simulink model "Autonomous_Microgrid_Test_backup"  (R2025b)
settings: Solver=FixedStepDiscrete  StartTime=0.0  StopTime=10.0  FixedStep=0.01  RelTol=1e-3  EnableMultiTasking=on
undefined symbols (not defined in the file): I_MAX, T_MAX, V_MAX, V_MIN
libraries: arduinolib x5
settings Model: ExtModeTrigDuration=2  Creator=Faculty  LastModifiedBy=Faculty
settings SolverCC: AutoInsertRateTranBlk=on
settings DataIOCC: ReturnWorkspaceOutputs=off
settings OptimizationCC: EnhancedBackFolding=on  PassReuseOutputArgsAs=Individual arguments  ZeroExternalMemoryAtStartup=off  ZeroInternalMemoryAtStartup=off  MaxStackSize=64  OptimizeBlockOrder=speed  DifferentSizesBufferReuse=on  OptimizationCustomize=off  EfficientTunableParamExpr=on
settings DebuggingCC: ParameterTunabilityLossMsg=error
settings HardwareCC: ProdBitPerPointer=32.0  ProdBitPerSizeT=32.0  ProdBitPerPtrDiffT=32.0  ProdLargestAtomicInteger=Long  ProdLargestAtomicFloat=Double  ProdWordSize=32.0  ProdHWDeviceType=ARM Compatible->ARM Cortex  UseEmbeddedCoderFeatures=off  UseSimulinkCoderFeatures=off
settings SFSimCC: MATLABDynamicMemAlloc=off
settings RTWCC: SystemTargetFile=ert.tlc  HardwareBoard=Arduino Uno R4 WiFi  TemplateMakefile=ert_default_tmf  Toolchain=Arduino ARM M4  BuildConfiguration=Faster Runs  Description=Embedded Coder
settings CodeAppCC: ForceParamTrailComments=on  IgnoreCustomStorageClasses=off  OperatorAnnotations=on  SimulinkDataObjDesc=on  SFDataObjDesc=on  InsertBlockDesc=on
settings ERTTargetCC: ExtModeTransport=3.0  ExtModeStaticAlloc=on  ExtModeAutomaticAllocSize=off  ExtModeStaticAllocSize=8192.0  ExtModeMexFile=ext_xcp  ExtModeIntrfLevel=Level2 - Open  InlinedParameterPlacement=Hierarchical  SupportContinuousTime=on  SupportNonInlinedSFcns=on  SupportVariableSizeSignals=on

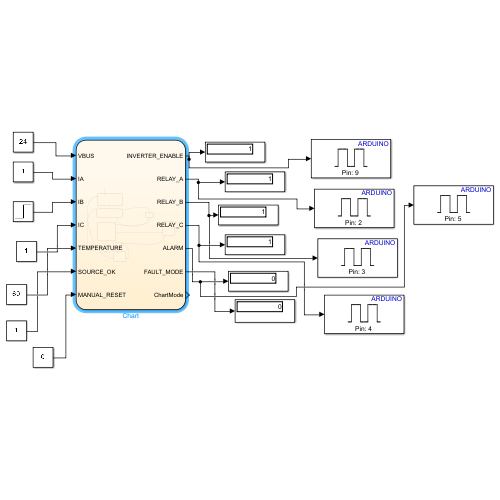
[thumbnail: Simulink's stored preview of the top-level diagram]
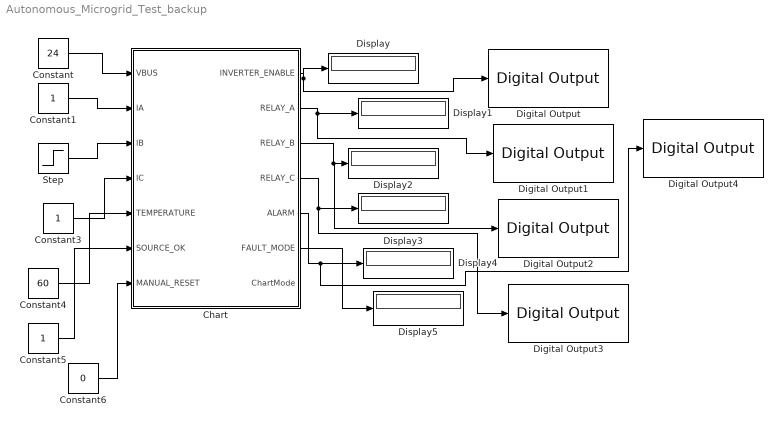
== system Autonomous_Microgrid_Test_backup ==
  Chart : Stateflow chart  TreatAsAtomicUnit=on
  Constant : Constant  Value=24
  Constant1 : Constant
  Constant3 : Constant
  Constant4 : Constant  Value=60
  Constant5 : Constant
  Constant6 : Constant  Value=0
  Digital Output : arduinolib/Digital Output  pinNumber=9  Direction=output  blockPlatform=arduino
  Digital Output1 : arduinolib/Digital Output  pinNumber=2  Direction=output  blockPlatform=arduino
  Digital Output2 : arduinolib/Digital Output  pinNumber=3  Direction=output  blockPlatform=arduino
  Digital Output3 : arduinolib/Digital Output  pinNumber=4  Direction=output  blockPlatform=arduino
  Digital Output4 : arduinolib/Digital Output  pinNumber=5  Direction=output  blockPlatform=arduino
  Display{,1..5} (6 alike) : Display
  Step : Step  Time=2  Before=1  After=2  SampleTime=0
  wires:
  Constant6/1 -> Chart/7(MANUAL_RESET)
  Constant3/1 -> Chart/4(IC)
  Constant4/1 -> Chart/5(TEMPERATURE)
  Constant5/1 -> Chart/6(SOURCE_OK)
  Step/1 -> Chart/3(IB)
  Constant1/1 -> Chart/2(IA)
  Constant/1 -> Chart/1(VBUS)
  Chart/1(INVERTER_ENABLE) -> Digital Output/1, Display/1
  Chart/2(RELAY_A) -> Digital Output1/1, Display1/1
  Chart/3(RELAY_B) -> Digital Output2/1, Display2/1
  Chart/4(RELAY_C) -> Digital Output3/1, Display3/1
  Chart/6(FAULT_MODE) -> Display5/1
  Chart/5(ALARM) -> Digital Output4/1, Display4/1

== stateflow chart Autonomous_Microgrid_Test_backup/Chart ==
  settings: updateMethod=DISCRETE  sampleTime=0.01
  state START_UP
    entry:
    INVERTER_ENABLE = false;
    RELAY_A = false;
    RELAY_B = false;
    RELAY_C = false;
    ALARM = false;
    FAULT_MODE = uint8(0);
  state NORMAL
    entry:
    INVERTER_ENABLE = true;
    RELAY_A = true;
    RELAY_B = true;
    RELAY_C = true;
    ALARM = false;
    FAULT_MODE = uint8(0);
  state WARNING
  state ISOLATE_FAULT
    entry:
    if FAULT_MODE == uint8(1)
    RELAY_A = false;
    elseif FAULT_MODE == uint8(2)
    RELAY_B = false;
    elseif FAULT_MODE == uint8(3)
    RELAY_C = false;
    else
    INVERTER_ENABLE = false;
    end
  state FAULT_DETECT
    entry:
    ALARM = true;
    if IA > I_MAX
    FAULT_MODE = uint8(1);
    elseif IB > I_MAX
    FAULT_MODE = uint8(2);
    elseif IC > I_MAX
    FAULT_MODE = uint8(3);
    elseif VBUS > V_MAX
    FAULT_MODE = uint8(4);
    elseif VBUS < V_MIN
    FAULT_MODE = uint8(5);
    elseif TEMPERATURE > T_MAX
    FAULT_MODE = uint8(6);
    elseif ~SOURCE_OK
    FAULT_MODE = uint8(7);
    end
  state SYSTEM_CHECK
  state RECOVERY
  state SHUTDOWN
    entry:
    INVERTER_ENABLE = false;
    RELAY_A = false;
    RELAY_B = false;
    RELAY_C = false;
    ALARM = true;
  (default) -> START_UP
  SHUTDOWN -> START_UP : [MANUAL_RESET]
  START_UP -> NORMAL : [SOURCE_OK && VBUS >= V_MIN && VBUS <= V_MAX]
  NORMAL -> WARNING : [IA > I_MAX || IB > I_MAX || IC > I_MAX || ...
      |  VBUS > V_MAX || VBUS < V_MIN || ...
      |  TEMPERATURE > T_MAX || ~SOURCE_OK]
  RECOVERY -> NORMAL : after(1,sec)
  WARNING -> FAULT_DETECT [order 1] : after(0.2,sec)
  WARNING -> NORMAL [order 2] : [IA <= I_MAX && IB <= I_MAX && IC <= I_MAX && ...
      |  VBUS >= V_MIN && VBUS <= V_MAX && ...
      |  TEMPERATURE <= T_MAX && SOURCE_OK]
  FAULT_DETECT -> ISOLATE_FAULT
  ISOLATE_FAULT -> SYSTEM_CHECK
  SYSTEM_CHECK -> SHUTDOWN [order 2] : [VBUS < V_MIN || VBUS > V_MAX || ...
      |  TEMPERATURE >= T_MAX || SOURCE_OK == 0]
  SYSTEM_CHECK -> RECOVERY [order 1] : [VBUS >= V_MIN && VBUS <= V_MAX && ...
      |  TEMPERATURE < T_MAX && SOURCE_OK == 1]
  data: VBUS input; IA input; IB input; IC input; TEMPERATURE input; SOURCE_OK input; MANUAL_RESET input; V_MAX parameter; V_MIN parameter; I_MAX parameter; T_MAX parameter; INVERTER_ENABLE output boolean size=1; RELAY_A output boolean size=1; RELAY_B output boolean size=1; RELAY_C output boolean size=1; ALARM output boolean size=1; FAULT_MODE output uint8 size=1; ChartMode output Enum: ChartModeType
